simulink model "Fractional"  (R2021b)
settings: Solver=ode45  StartTime=0.0  StopTime=1.6e-5  FixedStep=0.001/(2.56*2*synFr)  MaxStep=1/(25*synFr*synN)  RelTol=1e-5  AbsTol=1e-4  EnableMultiTasking=on
PreLoadFcn:
  | synFr=10e6; % Reference frequency
  | synFq=90e6; % VCO quiescent frequency
  | synSen=10e6; % VCO sensitivity
  | synN=10; % Fractional factor
  | synM=.3; % Fractional factor
undefined symbols (not defined in the file): Newton, Raphson
libraries: simulink_extras x5, dspstat3 x2, dspobslib x2, commsynccomp2 x1, simulink x1, dspsigops x1, dsparch4 x1
settings Model: Creator=The MathWorks, Inc.  LastModifiedBy=think
settings Model: ModifiedHistory=|
  | phase error compensation and swallow counter
  | incorporated by Benson,  Fall 2001.
settings SolverCC: AutoScaleAbsTol=off  AlgebraicLoopSolver=TrustRegion
settings DataIOCC: SaveFormat=Array  SaveOutput=off  SaveTime=off  ReturnWorkspaceOutputs=off  SignalLoggingName=sigsOut
settings OptimizationCC: BlockReduction=off  BooleanDataType=off  OptimizeBlockIOStorage=off  BufferReuse=off  GlobalBufferReuse=off  ExpressionFolding=off  ExpressionDepthLimit=2147483647  LocalBlockOutputs=off  InitFltsAndDblsToZero=on  LifeSpan=inf  OptimizeDataStoreBuffers=off  BusAssignmentInplaceUpdate=off
settings DebuggingCC: ReadBeforeWriteMsg=DisableAll  WriteAfterWriteMsg=DisableAll  WriteAfterReadMsg=DisableAll  SaveWithParameterizedLinksMsg=none  UnderspecifiedInitializationDetection=Classic  MergeDetectMultiDrivingBlocksExec=none  SignalResolutionControl=TryResolveAllWithWarning  MultiTaskDSMMsg=warning  MultiTaskCondExecSysMsg=none  FcnCallInpInsideContextMsg=warning  AllowSymbolicDim=off  StateNameClashWarn=warning  SFUnexpectedBacktrackingDiag=warning  SFNoUnconditionalDefaultTransitionDiag=warning  SFExecutionAtInitializationDiag=none  SFMachineParentedDataDiag=warning  ArithmeticOperatorsInVariantConditions=warning
settings HardwareCC: ProdBitPerPointer=32  ProdBitPerSizeT=32  ProdBitPerPtrDiffT=32  ProdLargestAtomicFloat=None  ProdIntDivRoundTo=Undefined  ProdEndianess=Unspecified  ProdWordSize=32  ProdHWDeviceType=32-bit Generic  TargetUnknown=on
settings ModelReferenceCC: PropagateSignalLabelsOutOfModel=off
settings SFSimCC: SimUseLocalCustomCode=off  CustomCodeUndefinedFunction=UseInterfaceOnly
settings RTWCC: RTWUseLocalCustomCode=off
settings CodeAppCC: StateflowObjectComments=on
settings GRTTargetCC: TargetFcnLib=ansi_tfl_tmw.mat  TargetLangStandard=C89/C90 (ANSI)  CombineOutputUpdateFcns=off  GRTInterface=on
settings ConfigComp: CovMetricSettings=dw  CovSaveCumulativeToWorkspaceVar=on  CovSaveSingleToWorkspaceVar=on  CovExternalEMLEnable=off  CovSFcnEnable=off

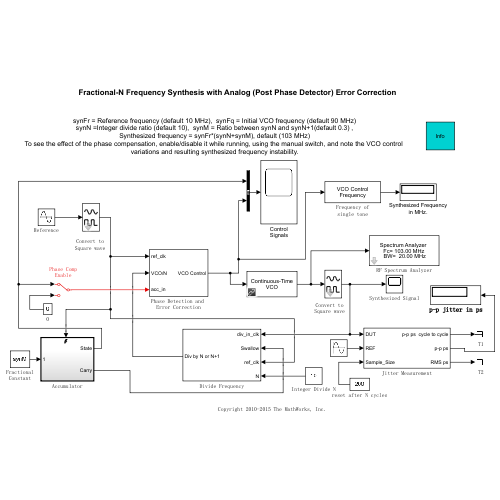
[thumbnail: Simulink's stored preview of the top-level diagram]
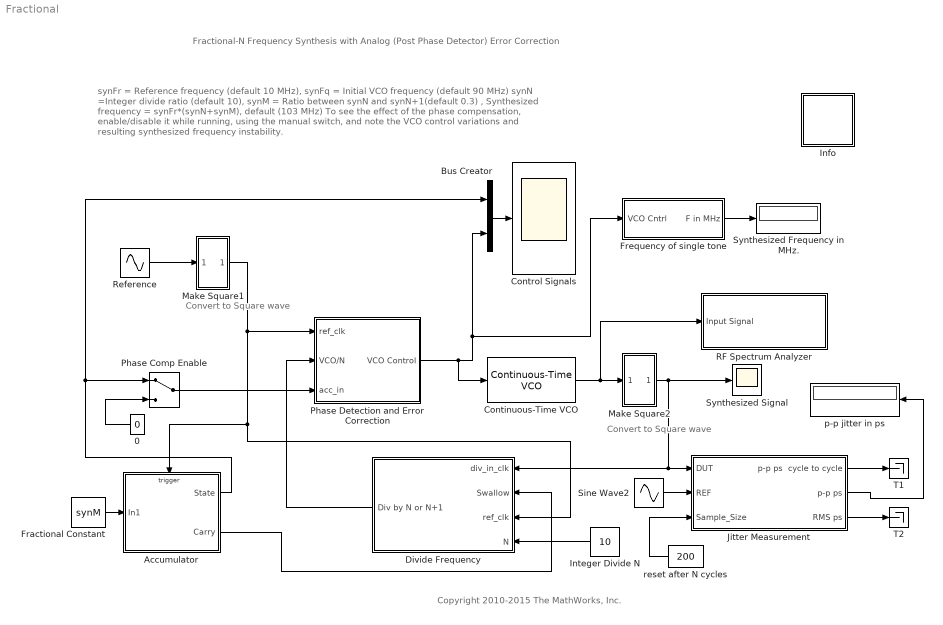
== system Fractional ==
  note: Convert to
      | Square wave
  note: Convert to
      | Square wave
  note: synFr = Reference frequency (default 10 MHz),  synFq = Initial VCO frequency (default 90 MHz)
      | synN =Integer divide ratio (default 10),  synM = Ratio between synN and synN+1(default 0.3) ,
      | Synthesized frequency = synFr*(synN+synM), default (103 MHz)
      | To see the effect of the phase compensation, enable/disable it while running, using the manual switch, and note the VCO control
      | variations and resulting synthesized frequency instability.
  note: Fractional-N Frequency Synthesis with Analog (Post Phase Detector) Error Correction
  note: Copyright 2010-2015 The MathWorks, Inc.
  0 : Constant  Value=0
  Accumulator : Subsystem  TreatAsAtomicUnit=on
  Bus Creator : BusCreator  Inputs=2
  Continuous-Time VCO : commsynccomp2/Continuous-Time VCO  Ac=1  Fc=synFq  Kc=synSen  Ph=0
      settings: SourceProductBaseCode=CM
  Control Signals : Scope
  Divide Frequency : Subsystem
  Fractional Constant : Constant  Value=synM
  Frequency of single tone : Subsystem
      mask Display: disp('VCO Control\nFrequency')
  Info : Subsystem  mask(Info){}
      settings: OpenFcn=web(commdhelp, '-helpbrowser');
      mask Display: disp('Info')
  Integer Divide N : Constant  Value=10
  Jitter Measurement : Subsystem
  Make Square1 : Subsystem  mask(Make Square){}
      mask help:
      | For input +ve values output is 1
      | For input -ve values output is 0
      mask Display: plot(0,0,100,100,[90,70,70,50,50,30,30,10,10],[20,20,40,40,20,20,40,40,20],[90,87,84,80,76,73,70,67,63,60,57,53,50,47,44,40,36,33,30,27,23,20,17,13,10],[70,65,63,62,63,65,70,75,77,78,77,75,70,65,63,62,63,65,70,75,77,78,77,75,70])
  Make Square2 : Subsystem  mask(Make Square){}
      mask help:
      | For input +ve values output is 1
      | For input -ve values output is 0
      mask Display: plot(0,0,100,100,[90,70,70,50,50,30,30,10,10],[20,20,40,40,20,20,40,40,20],[90,87,84,80,76,73,70,67,63,60,57,53,50,47,44,40,36,33,30,27,23,20,17,13,10],[70,65,63,62,63,65,70,75,77,78,77,75,70,65,63,62,63,65,70,75,77,78,77,75,70])
  Phase Comp Enable : ManualSwitch
  Phase Detection and Error Correction : Subsystem
  RF Spectrum Analyzer : Subsystem  Description=Spectrum Analyzer  mask{BW=synFr/.5 %20e6, Fc=synFr*(synM+synN)}
      mask prompts: BW "Bandwidth"; Fc "Center Freq"
      mask Display: fprintf('Spectrum Analyzer \n Fc=%7.2f MHz \n BW=%7.2f MHz',Fc/1e6,BW/1e6)
  Reference : Sin  Frequency=2*pi*synFr  Phase=pi  SampleTime=0
  Sine Wave2 : Sin  Frequency=2*pi*synFr*(synN+synM)  SampleTime=0
  Synthesized Frequency in MHz. : Display
      settings: Decimation=401
  Synthesized Signal : Scope
  T1 : Terminator
  T2 : Terminator
  p-p jitter in ps : Display
  reset after N cycles : Constant  Value=200  VectorParams1D=off
  wires:
  Divide Frequency/1(Div by N or N+1) -> Phase Detection and Error Correction/2(VCO/N)
  Fractional Constant/1 -> Accumulator/1(In1)
  Make Square2/1(Out1) -> Synthesized Signal/1, Divide Frequency/1(div_in_clk), Jitter Measurement/1(DUT)
  Accumulator/2(Carry) -> Divide Frequency/2(Swallow)
  Integer Divide N/1 -> Divide Frequency/4(N)
  0/1 -> Phase Comp Enable/2
  Frequency of single tone/1(F in MHz) -> Synthesized Frequency in MHz./1
  Sine Wave2/1 -> Jitter Measurement/2(REF)
  Jitter Measurement/2(p-p ps) -> p-p jitter in ps/1
  reset after N cycles/1 -> Jitter Measurement/3(Sample_Size)
  Bus Creator/1 -> Control Signals/1
  Accumulator/1(State) -> Bus Creator/1, Phase Comp Enable/1
  Make Square1/1(Out1) -> Accumulator/Trigger, Divide Frequency/3(ref_clk), Phase Detection and Error Correction/1(ref_clk)
  Phase Comp Enable/1 -> Phase Detection and Error Correction/3("acc_in ")
  Continuous-Time VCO/1 -> Make Square2/1(In1), RF Spectrum Analyzer/1(Input Signal)
  Phase Detection and Error Correction/1(VCO Control) -> Frequency of single tone/1(VCO Cntrl), Bus Creator/2, Continuous-Time VCO/1
  Reference/1 -> Make Square1/1(In1)
  Jitter Measurement/1(p-p ps  cycle to cycle) -> T1/1
  Jitter Measurement/3(RMS ps) -> T2/1

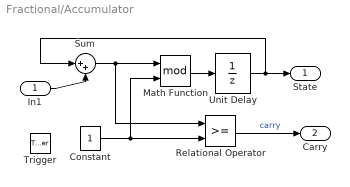
== system Fractional/Accumulator ==
  In1 : Inport
  Trigger : TriggerPort  VariantControl=Variant
  Constant : Constant
  Math Function : Math  Operator=mod  SignedPower=on  SaturateOnIntegerOverflow=on
  Relational Operator : RelationalOperator  RndMeth=Nearest  InputSameDT=on
  Sum : Sum  Inputs=|++  InputSameDT=on  SaturateOnIntegerOverflow=on  OutDataTypeStr=Inherit: Same as first input
  Unit Delay : UnitDelay  SampleTime=-1  HasFrameUpgradeWarning=on
  State : Outport  InitialOutput=0
  Carry : Outport  Port=2
  wires:
  In1/1 -> Sum/2
  Sum/1 -> Relational Operator/1, Math Function/1
  Math Function/1 -> Unit Delay/1
  Constant/1 -> Math Function/2, Relational Operator/2
  Relational Operator/1 -> Carry/1  "carry"
  Unit Delay/1 -> Sum/1, State/1

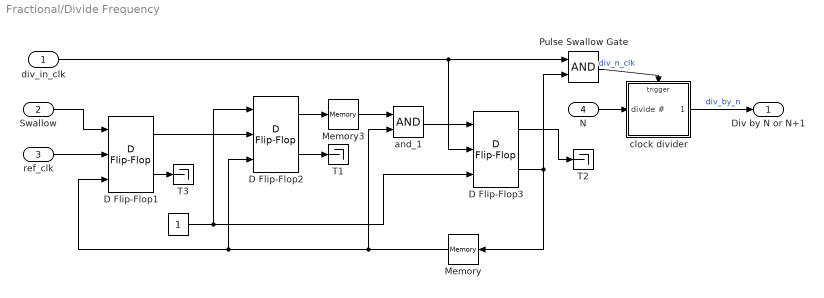
== system Fractional/Divide Frequency ==
  div_in_clk : Inport
  Swallow : Inport  Port=2
  ref_clk : Inport  Port=3
  N : Inport  Port=4
  " " : Constant
  D Flip-Flop1 : simulink_extras/Flip Flops/D Flip-Flop
  D Flip-Flop2 : simulink_extras/Flip Flops/D Flip-Flop
  D Flip-Flop3 : simulink_extras/Flip Flops/D Flip-Flop
  Memory : Memory
  Memory3 : Memory
  Pulse Swallow Gate : Logic
  T1 : Terminator
  T2 : Terminator
  T3 : Terminator
  and_1 : Logic
  clock divider : Subsystem  TreatAsAtomicUnit=on
  Div by N or N+1 : Outport
  wires:
  N/1 -> clock divider/1("divide # ")
  D Flip-Flop1/2 -> T3/1
  D Flip-Flop2/2 -> T1/1
  D Flip-Flop3/1 -> T2/1
  Memory3/1 -> and_1/1
  D Flip-Flop1/1 -> D Flip-Flop2/2
  ref_clk/1 -> D Flip-Flop1/2
  Swallow/1 -> D Flip-Flop1/1
  and_1/1 -> D Flip-Flop3/1
  " "/1 -> D Flip-Flop3/3, D Flip-Flop2/1
  Memory/1 -> and_1/2, D Flip-Flop1/3, D Flip-Flop2/3
  D Flip-Flop3/2 -> Memory/1, Pulse Swallow Gate/2
  D Flip-Flop2/1 -> Memory3/1
  div_in_clk/1 -> D Flip-Flop3/2, Pulse Swallow Gate/1
  clock divider/1(" ") -> Div by N or N+1/1  "div_by_n"
  Pulse Swallow Gate/1 -> clock divider/Trigger  "div_n_clk"

== system Fractional/Frequency of single tone ==
  VCO Cntrl : Inport
  F : Constant  Value=synFq
  Gain3 : Gain  Gain=synSen  SaturateOnIntegerOverflow=on  OutDataTypeStr=Inherit: Same as input  ParamDataTypeStr=Inherit: Same as input
  Sum1 : Sum  Inputs=|++  InputSameDT=on  SaturateOnIntegerOverflow=on  OutDataTypeStr=Inherit: Same as first input
  F in MHz : Outport
  wires:
  F/1 -> Sum1/2
  Gain3/1 -> Sum1/1
  VCO Cntrl/1 -> Gain3/1
  Sum1/1 -> F in MHz/1

== system Fractional/Info ==

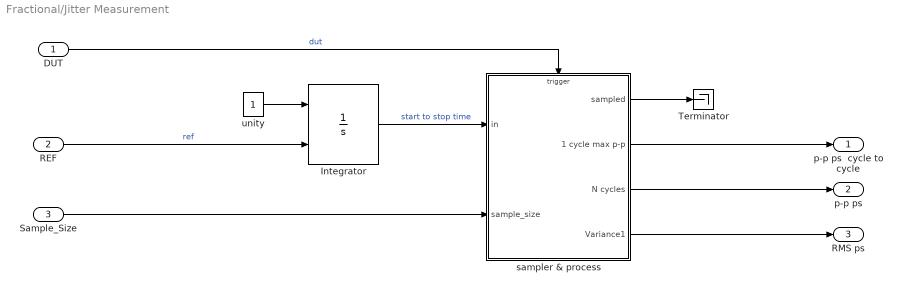
== system Fractional/Jitter Measurement ==
  DUT : Inport
  REF : Inport  Port=2
  Sample_Size : Inport  Port=3
  Integrator : Integrator  ExternalReset=rising
  Terminator : Terminator
  sampler & process : Subsystem  TreatAsAtomicUnit=on
  unity : Constant  OutDataTypeStr=double
  p-p ps  cycle to cycle : Outport
  p-p ps : Outport  Port=2
  RMS ps : Outport  Port=3
  wires:
  DUT/1 -> sampler & process/Trigger  "dut"
  REF/1 -> Integrator/2  "ref"
  Integrator/1 -> sampler & process/1(in)  "start to stop time"
  Sample_Size/1 -> sampler & process/2(sample_size)
  sampler & process/3(N cycles) -> p-p ps/1
  sampler & process/4(Variance1) -> RMS ps/1
  unity/1 -> Integrator/1
  sampler & process/2(1 cycle max p-p) -> p-p ps  cycle to cycle/1
  sampler & process/1(sampled) -> Terminator/1

== system Fractional/Make Square1 ==
  In1 : Inport
  Constant : Constant  Value=0
  Relational Operator : RelationalOperator  Operator=>  RndMeth=Nearest  InputSameDT=on
  Out1 : Outport
  wires:
  In1/1 -> Relational Operator/1
  Constant/1 -> Relational Operator/2
  Relational Operator/1 -> Out1/1

== system Fractional/Make Square2 ==
  In1 : Inport
  Constant : Constant  Value=0
  Relational Operator : RelationalOperator  Operator=>  RndMeth=Nearest  InputSameDT=on
  Out1 : Outport
  wires:
  Relational Operator/1 -> Out1/1
  Constant/1 -> Relational Operator/2
  In1/1 -> Relational Operator/1

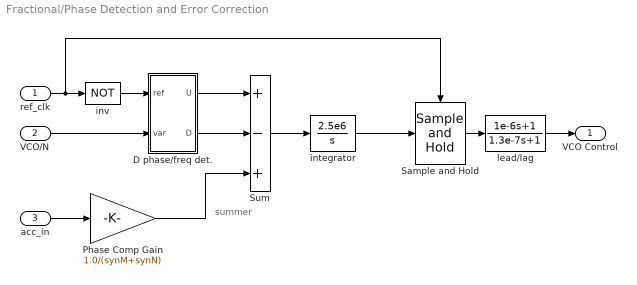
== system Fractional/Phase Detection and Error Correction ==
  note: summer
  ref_clk : Inport
  VCO/N : Inport  Port=2
  "acc_in " : Inport  Port=3
  "D phase/freq det. " : Subsystem
  Phase Comp Gain : Gain  Gain=1.0/(synM+synN)  SaturateOnIntegerOverflow=on  OutDataTypeStr=Inherit: Same as input  ParamDataTypeStr=Inherit: Same as input
  Sample and Hold : dspsigops/Sample and Hold  trig=Rising edge  initCond=0  latchinput=off
  Sum : Sum  Inputs=+-+  InputSameDT=on  SaturateOnIntegerOverflow=on  OutDataTypeStr=Inherit: Same as first input
  integrator : TransferFcn  Numerator=[2.5e6]  Denominator=[1 0]
  inv : Logic  Operator=NOT
  lead/lag : TransferFcn  Numerator=[1e-6 1]  Denominator=[1.3e-7 1]
  VCO Control : Outport
  wires:
  "D phase/freq det. "/1(U) -> Sum/1
  "D phase/freq det. "/2(D) -> Sum/2
  Sum/1 -> integrator/1
  inv/1 -> "D phase/freq det. "/1(ref)
  ref_clk/1 -> inv/1, Sample and Hold/Trigger
  VCO/N/1 -> "D phase/freq det. "/2(var)
  lead/lag/1 -> VCO Control/1
  "acc_in "/1 -> Phase Comp Gain/1
  Phase Comp Gain/1 -> Sum/3
  Sample and Hold/1 -> lead/lag/1
  integrator/1 -> Sample and Hold/1

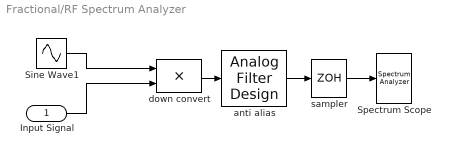
== system Fractional/RF Spectrum Analyzer ==
  Input Signal : Inport
  Sine Wave1 : Sin  Amplitude=1/3.6  Frequency=2*pi*(Fc-BW/2)  Phase=-pi/2  SampleTime=0
  Spectrum Scope : SpectrumAnalyzer
  anti alias : dsparch4/Analog Filter Design  method=Elliptic  filttype=Lowpass  N=8  Wlo=BW*2*pi  Whi=80  Rp=0.11  Rs=100
  down convert : Product  InputSameDT=on  SaturateOnIntegerOverflow=on  OutDataTypeStr=Inherit: Same as first input
  sampler : ZeroOrderHold  SampleTime=1/(2.56*BW)
  wires:
  Sine Wave1/1 -> down convert/1
  sampler/1 -> Spectrum Scope/1
  anti alias/1 -> sampler/1
  down convert/1 -> anti alias/1
  Input Signal/1 -> down convert/2

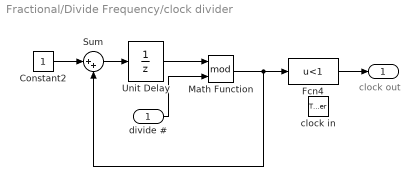
== system Fractional/Divide Frequency/clock divider ==
  note: clock out
  "divide # " : Inport
  clock in : TriggerPort  VariantControl=Variant
  Constant2 : Constant
  Fcn4 : Fcn  Expr=u<1
  Math Function : Math  Operator=mod  SignedPower=on  SaturateOnIntegerOverflow=on
  Sum : Sum  Inputs=|++  InputSameDT=on  SaturateOnIntegerOverflow=on  OutDataTypeStr=Inherit: Same as first input
  Unit Delay : UnitDelay  SampleTime=-1  HasFrameUpgradeWarning=on
  " " : Outport
  wires:
  "divide # "/1 -> Math Function/2
  Fcn4/1 -> " "/1
  Math Function/1 -> Fcn4/1, Sum/2
  Unit Delay/1 -> Math Function/1
  Constant2/1 -> Sum/1
  Sum/1 -> Unit Delay/1

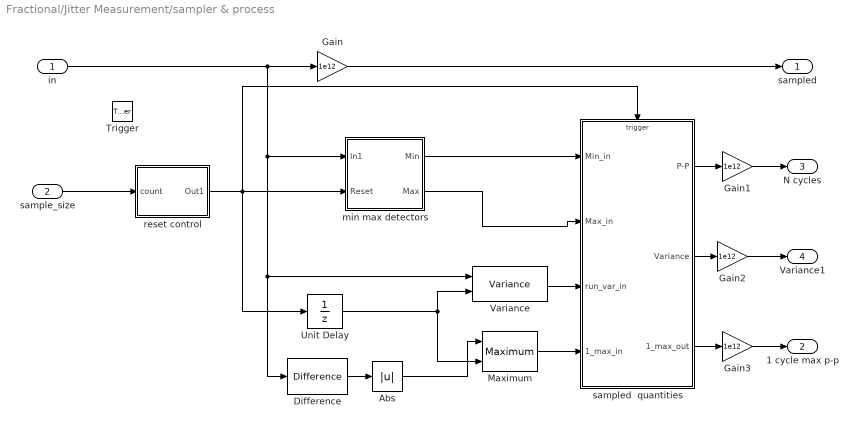
== system Fractional/Jitter Measurement/sampler & process ==
  in : Inport
  sample_size : Inport  Port=2
  Trigger : TriggerPort  VariantControl=Variant
  Abs : Abs
  Difference : simulink/Discrete/Difference  ICPrevInput=0.0  OutMin=[]  OutMax=[]  OutDataType=sfix(16)  OutScaling=2^-10  DoSatur=off
  Gain{,1..3} (4 alike) : Gain  Gain=1e12
  Maximum : dspstat3/Maximum  operation=maximum  fcn=Running  indexBase=One  operateOver=Each column  Dimension=1  reset=Rising edge  roiEnable=off  roiType=Rectangles  roiPortion=Entire ROI  roiOutput=Individual statistics for each ROI  roiFlag=off  roundingMode=Floor  overflowMode=off  accumDataTypeStr=Inherit: Same as product output  accumLastDataTypeStr=Inherit: Same as product output
  Unit Delay : UnitDelay  SampleTime=-1  HasFrameUpgradeWarning=on
  Variance : dspstat3/Variance  run=on  reset_popup=Rising edge  directionMode=Each column  dimension=1  roiEnable=off  roiType=Rectangles  roiPortion=Entire ROI  roiOutput=Individual statistics for each ROI  roiFlag=off  roundingMode=Floor  overflowMode=off
  min max detectors : Subsystem
  reset control : Subsystem
  sampled  quantities : Subsystem  TreatAsAtomicUnit=on
  sampled : Outport
  1 cycle max p-p : Outport  Port=2
  N cycles : Outport  Port=3
  Variance1 : Outport  Port=4
  wires:
  in/1 -> Gain/1, Variance/1, Difference/1, min max detectors/1(In1)
  Difference/1 -> Abs/1
  Abs/1 -> Maximum/1
  sample_size/1 -> reset control/1(count)
  reset control/1(Out1) -> Unit Delay/1, sampled  quantities/Trigger, min max detectors/2(Reset)
  sampled  quantities/1(P-P) -> Gain1/1
  Variance/1 -> sampled  quantities/3(run_var_in)
  sampled  quantities/2(Variance) -> Gain2/1
  Unit Delay/1 -> Variance/2, Maximum/2
  Maximum/1 -> sampled  quantities/4(1_max_in)
  sampled  quantities/3(1_max_out) -> Gain3/1
  Gain/1 -> sampled/1
  Gain1/1 -> N cycles/1
  Gain2/1 -> Variance1/1
  Gain3/1 -> 1 cycle max p-p/1
  min max detectors/2(Max) -> sampled  quantities/2(Max_in)
  min max detectors/1(Min) -> sampled  quantities/1(Min_in)

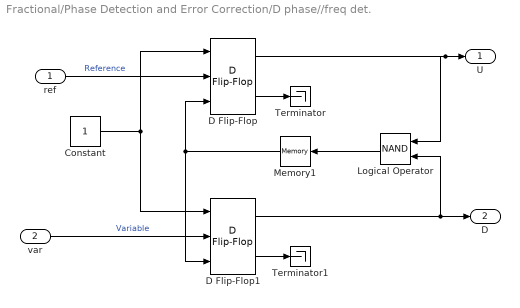
== system Fractional/Phase Detection and Error Correction/D phase//freq det.  ==
  ref : Inport
  var : Inport  Port=2
  Constant : Constant
  D Flip-Flop : simulink_extras/Flip Flops/D Flip-Flop
  D Flip-Flop1 : simulink_extras/Flip Flops/D Flip-Flop
  Logical Operator : Logic  Operator=NAND
  Memory1 : Memory
  Terminator : Terminator
  Terminator1 : Terminator
  U : Outport
  D : Outport  Port=2
  wires:
  var/1 -> D Flip-Flop1/2  "Variable"
  D Flip-Flop/2 -> Terminator/1
  D Flip-Flop1/2 -> Terminator1/1
  ref/1 -> D Flip-Flop/2  "Reference"
  Constant/1 -> D Flip-Flop/1, D Flip-Flop1/1
  Memory1/1 -> D Flip-Flop/3, D Flip-Flop1/3
  D Flip-Flop/1 -> U/1, Logical Operator/1
  D Flip-Flop1/1 -> D/1, Logical Operator/2
  Logical Operator/1 -> Memory1/1

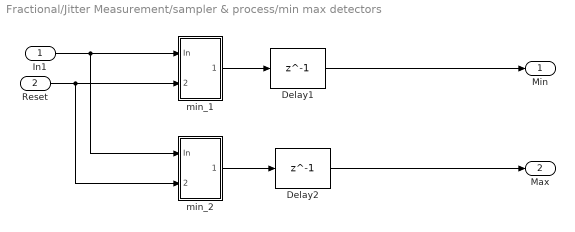
== system Fractional/Jitter Measurement/sampler & process/min max detectors ==
  In1 : Inport
  Reset : Inport  Port=2
  Delay1 : Delay  DelayLength=1  InitialCondition=0  UseCircularBuffer=on
  Delay2 : Delay  DelayLength=1  InitialCondition=0  UseCircularBuffer=on
  min_1 : Subsystem
  min_2 : Subsystem
  Min : Outport
  Max : Outport  Port=2
  wires:
  Reset/1 -> min_1/2(Rst), min_2/2(Rst)
  In1/1 -> min_1/1(In), min_2/1(In)
  min_1/1(Out) -> Delay1/1
  min_2/1(Out) -> Delay2/1
  Delay1/1 -> Min/1
  Delay2/1 -> Max/1

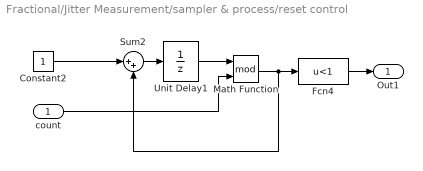
== system Fractional/Jitter Measurement/sampler & process/reset control ==
  count : Inport
  Constant2 : Constant
  Fcn4 : Fcn  Expr=u<1
  Math Function : Math  Operator=mod  SignedPower=on  SaturateOnIntegerOverflow=on
  Sum2 : Sum  Inputs=|++  InputSameDT=on  SaturateOnIntegerOverflow=on  OutDataTypeStr=Inherit: Same as first input
  Unit Delay1 : UnitDelay  SampleTime=-1  HasFrameUpgradeWarning=on
  Out1 : Outport
  wires:
  Math Function/1 -> Fcn4/1, Sum2/2
  Unit Delay1/1 -> Math Function/1
  Constant2/1 -> Sum2/1
  Sum2/1 -> Unit Delay1/1
  Fcn4/1 -> Out1/1
  count/1 -> Math Function/2

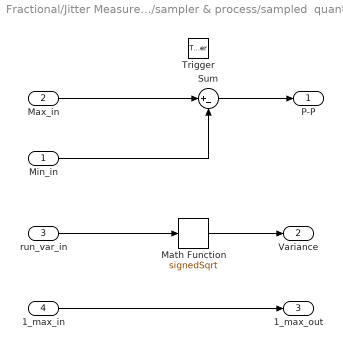
== system Fractional/Jitter Measurement/sampler & process/sampled  quantities ==
  Min_in : Inport
  Max_in : Inport  Port=2
  run_var_in : Inport  Port=3
  1_max_in : Inport  Port=4
  Trigger : TriggerPort  VariantControl=Variant
  Math Function : Sqrt  Operator=signedSqrt  AlgorithmType=Newton-Raphson  SaturateOnIntegerOverflow=on
  Sum : Sum  Inputs=|+-  InputSameDT=on  SaturateOnIntegerOverflow=on  OutDataTypeStr=Inherit: Same as first input
  P-P : Outport
  Variance : Outport  Port=2
  1_max_out : Outport  Port=3
  wires:
  Max_in/1 -> Sum/1
  Min_in/1 -> Sum/2
  Sum/1 -> P-P/1
  Math Function/1 -> Variance/1
  run_var_in/1 -> Math Function/1
  1_max_in/1 -> 1_max_out/1

== system Fractional/Jitter Measurement/sampler & process/min max detectors/min_1 ==
  In : Inport
  Rst : Inport  Port=2
  Delay : dspobslib/Delay  InputProcessing=Columns as channels (frame based)  dly_unit=Samples  delay=1  ic_detail=off  dif_ic_for_ch=off  dif_ic_for_dly=off  ic=1e6  reset_popup=Non-zero sample
      settings: SourceProductBaseCode=DS
  Relational Operator : RelationalOperator  Operator=<  OutDataTypeStr=boolean  RndMeth=Nearest
  Switch : Switch  Threshold=.5
  Out : Outport
  wires:
  In/1 -> Relational Operator/1, Switch/1
  Rst/1 -> Delay/2
  Delay/1 -> Relational Operator/2, Switch/3
  Relational Operator/1 -> Switch/2
  Switch/1 -> Delay/1, Out/1

== system Fractional/Jitter Measurement/sampler & process/min max detectors/min_2 ==
  In : Inport
  Rst : Inport  Port=2
  Delay : dspobslib/Delay  InputProcessing=Columns as channels (frame based)  dly_unit=Samples  delay=1  ic_detail=off  dif_ic_for_ch=off  dif_ic_for_dly=off  ic=-1e6  reset_popup=Non-zero sample
      settings: SourceProductBaseCode=DS
  Relational Operator : RelationalOperator  Operator=>  OutDataTypeStr=boolean  RndMeth=Nearest
  Switch : Switch  Threshold=.5
  Out : Outport
  wires:
  Switch/1 -> Out/1, Delay/1
  Relational Operator/1 -> Switch/2
  Delay/1 -> Switch/3, Relational Operator/2
  Rst/1 -> Delay/2
  In/1 -> Switch/1, Relational Operator/1
